simulink model "sl_pursuit2"  (R2019b)
settings: Solver=ode45  StartTime=0.0  StopTime=Inf  FixedStep=0.2  MaxStep=0.1  RelTol=1e-3  EnableMultiTasking=on
StartFcn:
  | % remove the red dashed line draw in StopFcn
  | set(0, 'ShowHiddenHandles', 'on')
  | h = findobj('Tag',  'SL_PURSUIT_PATH');
  | if ~isempty(h)
  |     delete(h)
  | end
  | set(0, 'ShowHiddenHandles', 'off')
StopFcn:
  | % get the waypoints from trajectory block
  | h = getSimulinkBlockHandle([gcs '/pure pursuit'])
  | path = str2num(get_param(h, 'path'));
  | 
  | % overlay it on the XY scope, tag it so it can be cleaned up in StartFcn
  | set(0, 'ShowHiddenHandles', 'on')
  | fig = findobj('name', 'XY');
  | ax = findobj('type', 'axes');
  | axes(ax);
  | hold on
  | plot(path(:,1), path(:,2), 'Color',  'red', 'LineStyle', '--', 'LineWidth', 2, 'Tag', 'SL_PURSUIT_PATH')
  | grid on
  | hold off
  | set(0, 'ShowHiddenHandles', 'off')
libraries: roblocks x3, simulink x2
settings Model: Creator=pic  LastModifiedBy=corkep
settings DataIOCC: SaveFormat=Array  SignalLoggingSaveFormat=ModelDataLogs  TimeSaveName=t  OutputSaveName=y
settings OptimizationCC: ExpressionDepthLimit=2147483647  LifeSpan=inf
settings DebuggingCC: UnderspecifiedInitializationDetection=Classic  MergeDetectMultiDrivingBlocksExec=none  SolverPrmCheckMsg=warning  FcnCallInpInsideContextMsg=warning  AllowSymbolicDim=off  StateNameClashWarn=warning  PregeneratedLibrarySubsystemCodeDiagnostic=none  SFUnexpectedBacktrackingDiag=warning  SFNoUnconditionalDefaultTransitionDiag=warning  SFExecutionAtInitializationDiag=none  ArithmeticOperatorsInVariantConditions=warning
settings HardwareCC: ProdBitPerPointer=32  ProdBitPerSizeT=32  ProdBitPerPtrDiffT=32  ProdLargestAtomicFloat=None  ProdIntDivRoundTo=Undefined  ProdEndianess=Unspecified  ProdWordSize=32  ProdHWDeviceType=32-bit Generic
settings ModelReferenceCC: PropagateSignalLabelsOutOfModel=off
settings SFSimCC: SimUseLocalCustomCode=off  CustomCodeUndefinedFunction=UseInterfaceOnly
settings RTWCC: RTWUseLocalCustomCode=off
settings CodeAppCC: StateflowObjectComments=on
settings GRTTargetCC: TargetLangStandard=C89/C90 (ANSI)  GeneratePreprocessorConditionals=Disable all  CombineOutputUpdateFcns=off  GRTInterface=on
settings ConfigComp: CovMetricSettings=dw  CovHtmlReporting=on  CovSaveCumulativeToWorkspaceVar=on  CovSaveSingleToWorkspaceVar=on  CovExternalEMLEnable=off

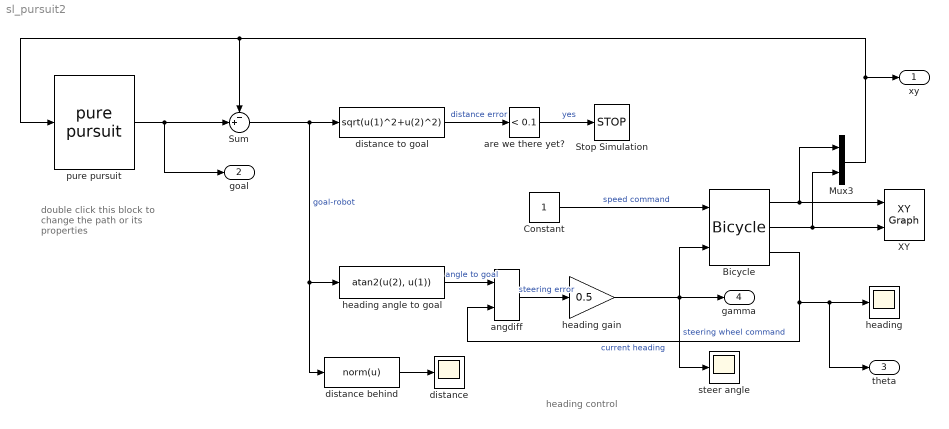
== system sl_pursuit2 ==
  note: heading control
  note: double click this block to
      | change the path or its
      | properties
  Bicycle : roblocks/Vehicles/Bicycle  vlim=5  accel=1  alim=0.5  steer_rate=Inf  L=1  x0=[0, 0, 0]
  Constant : Constant
  Mux3 : Mux  Inputs=2
  Stop Simulation : Stop
  Sum : Sum  Inputs=-+|
  XY : simulink/Sinks/XY Graph  xmin=0  xmax=100  ymin=0  ymax=100  st=-1
  angdiff : roblocks/Toolbox/angdiff
  are we there yet? : simulink/Logic and Bit Operations/Compare To Constant  relop=<  const=0.1  OutDataTypeStr=boolean
  distance : Scope
  distance behind : MATLABFcn  MATLABFcn=norm(u)
  distance to goal : Fcn  Expr=sqrt(u(1)^2+u(2)^2)
  "heading " : Scope
  heading angle to goal : Fcn  Expr=atan2(u(2), u(1))
  heading gain : Gain  Gain=0.5
  pure pursuit : roblocks/Toolbox/pure pursuit  path=|  vaxis=[2.5 2.5]  tseg=[]  dt=0.1  tacc=0  R=5
      | [  10 10;
      |   10 60;
      |   80 80;
      |   50 10 ]
  steer angle : Scope
  xy : Outport  VectorParamsAs1DForOutWhenUnconnected=off
  goal : Outport  Port=2  VectorParamsAs1DForOutWhenUnconnected=off
  theta : Outport  Port=3  VectorParamsAs1DForOutWhenUnconnected=off
  gamma : Outport  Port=4  VectorParamsAs1DForOutWhenUnconnected=off
  wires:
  Bicycle/1 -> Mux3/1, XY/1
  Bicycle/2 -> Mux3/2, XY/2
  Sum/1 -> distance behind/1, heading angle to goal/1, distance to goal/1  "goal-robot"
  heading angle to goal/1 -> angdiff/1  "angle to goal"
  Bicycle/3 -> theta/1, "heading "/1, angdiff/2  "current heading"
  angdiff/1 -> heading gain/1  "steering error"
  heading gain/1 -> gamma/1, Bicycle/2, steer angle/1  "steering wheel command"
  Constant/1 -> Bicycle/1  "speed command"
  distance behind/1 -> distance/1
  distance to goal/1 -> are we there yet?/1  "distance error"
  Mux3/1 -> pure pursuit/1, Sum/1, xy/1
  pure pursuit/1 -> goal/1, Sum/2
  are we there yet?/1 -> Stop Simulation/1  "yes"
